simulink model "LabPsu_discretePlant"  (R2026b)
values from neighbouring files (symbols this model uses):
  C = double(C)    [labpsu_discrete_plant_coeffs.m]    (also in plant.sldd = 0.0001)
  L = double(L)    [labpsu_discrete_plant_coeffs.m]    (also in plant.sldd = 1.0E-5)
  R = double(R)    [labpsu_discrete_plant_coeffs.m]    (also in plant.sldd = 5.0)
  RL = double(RL)    [labpsu_discrete_plant_coeffs.m]    (also in plant.sldd = 0.001)
  Vin = double(Vin)    [labpsu_discrete_plant_coeffs.m]    (also in plant.sldd = 24.0)
undefined symbols (not defined in the file or in its folder): dspblkCoreblockFVToolHelper, gcbh
settings Model: Creator=BenjaminRupp  LastModifiedBy=BenjaminRupp

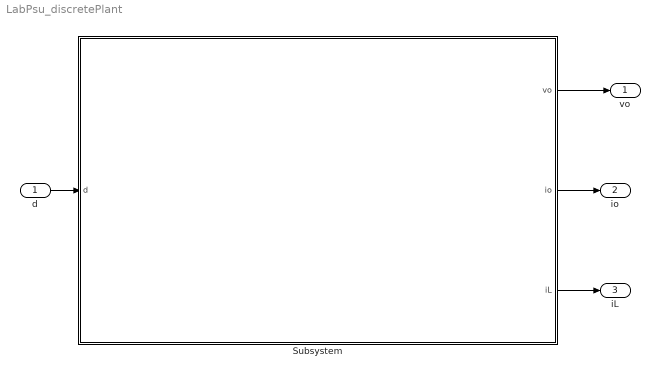
== system LabPsu_discretePlant ==
  d : Inport  OutDataTypeStr=single
  Subsystem : Subsystem  mask{L=L, R=R, Vin=Vin, RL=RL, C=C, Ts=1/10e3}
      mask init:
      | LabPsuDiscretePlant = labpsu_discrete_plant_coeffs(L, C, R, RL, Vin, Ts);
  vo : Outport  OutDataTypeStr=single
  io : Outport  Port=2  OutDataTypeStr=single
  iL : Outport  Port=3  OutDataTypeStr=single
  wires:
  d/1 -> Subsystem/1(d)
  Subsystem/1(vo) -> vo/1
  Subsystem/2(io) -> io/1
  Subsystem/3(iL) -> iL/1

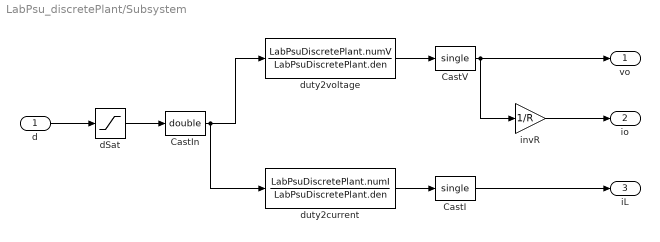
== system LabPsu_discretePlant/Subsystem ==
  d : Inport
  CastI : DataTypeConversion  OutDataTypeStr=single  SaturateOnIntegerOverflow=off  RndMeth=Floor
  CastIn : DataTypeConversion  OutDataTypeStr=double  SaturateOnIntegerOverflow=off  RndMeth=Floor
  CastV : DataTypeConversion  OutDataTypeStr=single  SaturateOnIntegerOverflow=off  RndMeth=Floor
  dSat : Saturate  UpperLimit=1  LowerLimit=0
  duty2current : DiscreteTransferFcn  LoadFcn=dspblkCoreblockFVToolHelper(gcbh,'load');  Numerator=LabPsuDiscretePlant.numI  Denominator=LabPsuDiscretePlant.den
      settings: CopyFcn=dspblkCoreblockFVToolHelper(gcbh,'copy');  DeleteFcn=dspblkCoreblockFVToolHelper(gcbh,'close');  ModelCloseFcn=dspblkCoreblockFVToolHelper(gcbh,'close');  PreSaveFcn=dspblkCoreblockFVToolHelper(gcbh,'presave');  PostSaveFcn=dspblkCoreblockFVToolHelper(gcbh,'postsave');  CloseFcn=dspblkCoreblockFVToolHelper(gcbh,'close');
  duty2voltage : DiscreteTransferFcn  LoadFcn=dspblkCoreblockFVToolHelper(gcbh,'load');  Numerator=LabPsuDiscretePlant.numV  Denominator=LabPsuDiscretePlant.den
      settings: CopyFcn=dspblkCoreblockFVToolHelper(gcbh,'copy');  DeleteFcn=dspblkCoreblockFVToolHelper(gcbh,'close');  ModelCloseFcn=dspblkCoreblockFVToolHelper(gcbh,'close');  PreSaveFcn=dspblkCoreblockFVToolHelper(gcbh,'presave');  PostSaveFcn=dspblkCoreblockFVToolHelper(gcbh,'postsave');  CloseFcn=dspblkCoreblockFVToolHelper(gcbh,'close');
  invR : Gain  Gain=1/R  OutDataTypeStr=single
  vo : Outport
  io : Outport  Port=2
  iL : Outport  Port=3
  wires:
  d/1 -> dSat/1
  CastV/1 -> vo/1, invR/1
  duty2current/1 -> CastI/1
  CastIn/1 -> duty2voltage/1, duty2current/1
  CastI/1 -> iL/1
  duty2voltage/1 -> CastV/1
  invR/1 -> io/1
  dSat/1 -> CastIn/1
